simulink model "blance_leg2_RPY"  (R2023a)
settings: Solver=VariableStepAuto  StartTime=0.0  StopTime=10  MaxStep=0.0050000000000000001  RelTol=5.0000000000000002e-05  AbsTol=9.9999999999999995e-07
InitFcn:
  | addpath(fileparts(get_param(bdroot,'FileName')));
  | apply_config(bdroot);
model workspace (MAT data in the model file):
  L_length_ref : timeseries (value not decoded)
  L_v_ref : timeseries (value not decoded)
  R_length_ref : timeseries (value not decoded)
  R_v_ref : timeseries (value not decoded)
  runScenario_cfg_override = []
  wheel_speed_compensation = 1
values from neighbouring files (symbols this model uses):
  K = cachedK    [configured_lqr_gain.m]    (also in get_k_length.m = lqr(A,B,Q,R); matlab.mat = [-1.73670717704  -0.157075032659  -0.691811333866  -0.787613)
  N = NM + mp*diff(x + L*sin(theta),t,2)    [get_k_length.m]
  s = sin(phi3 - phi2)    [five_bar_geometry_rm.m]
undefined symbols (not defined in the file or in its folder): X, Y, Z
libraries: sm_lib x82, nesl_utility x35, slpidlib x2
(part 3 of 3)

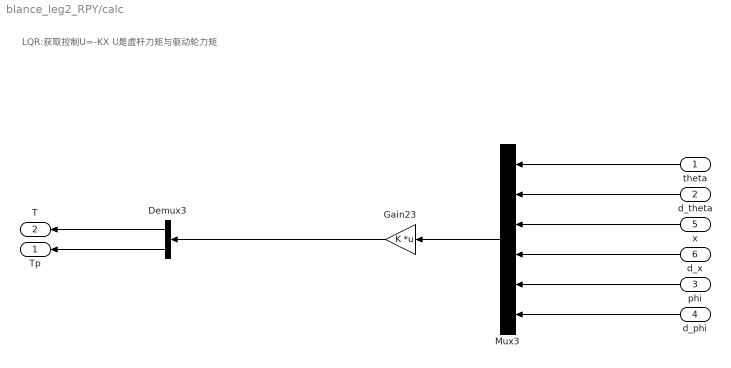
== system blance_leg2_RPY/calc ==
  note: LQR:获取控制U=-KX
      | U是虚杆力矩与驱动轮力矩
  theta : Inport
  d_theta : Inport  Port=2
  phi : Inport  Port=3
  d_phi : Inport  Port=4
  x : Inport  Port=5
  d_x : Inport  Port=6
  Demux3 : Demux  Outputs=2
  Gain23 : Gain  Gain=K  Multiplication=Matrix(K*u) (u vector)
  Mux3 : Mux  Inputs=6
  Tp : Outport
  T : Outport  Port=2
  wires:
  Demux3/1 -> T/1
  Demux3/2 -> Tp/1
  Mux3/1 -> Gain23/1
  theta/1 -> Mux3/1
  d_theta/1 -> Mux3/2
  x/1 -> Mux3/3
  d_x/1 -> Mux3/4
  phi/1 -> Mux3/5
  d_phi/1 -> Mux3/6
  Gain23/1 -> Demux3/1

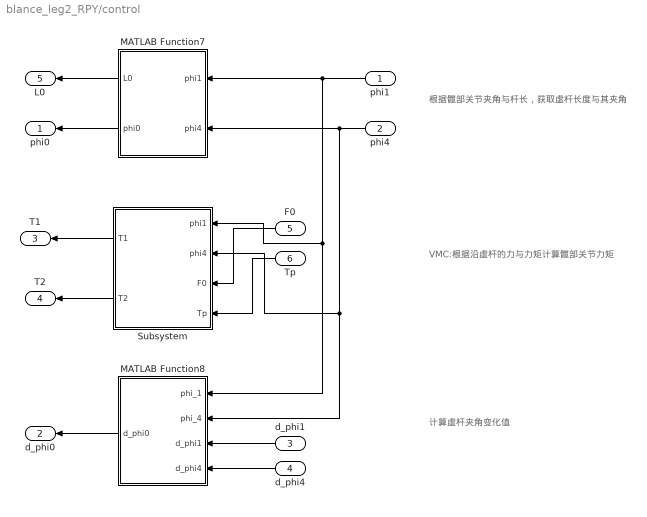
== system blance_leg2_RPY/control ==
  note: 计算虚杆夹角变化值
  note: VMC:根据沿虚杆的力与力矩计算髋部关节力矩
  note: 根据髋部关节夹角与杆长，获取虚杆长度与其夹角
  phi1 : Inport
  phi4 : Inport  Port=2
  d_phi1 : Inport  Port=3
  d_phi4 : Inport  Port=4
  F0 : Inport  Port=5
  Tp : Inport  Port=6
  MATLAB Function7 : MATLAB Function  TreatAsAtomicUnit=on
  MATLAB Function8 : MATLAB Function  TreatAsAtomicUnit=on
  Subsystem : Subsystem
  phi0 : Outport
  d_phi0 : Outport  Port=2
  T1 : Outport  Port=3
  T2 : Outport  Port=4
  L0 : Outport  Port=5
  wires:
  MATLAB Function7/2(phi0) -> phi0/1
  MATLAB Function8/1(d_phi0) -> d_phi0/1
  d_phi4/1 -> MATLAB Function8/4(d_phi4)
  d_phi1/1 -> MATLAB Function8/3(d_phi1)
  MATLAB Function7/1(L0) -> L0/1
  phi4/1 -> MATLAB Function7/2(phi4), Subsystem/2(phi4), MATLAB Function8/2(phi_4)
  phi1/1 -> MATLAB Function7/1(phi1), MATLAB Function8/1(phi_1), Subsystem/1(phi1)
  F0/1 -> Subsystem/3(F0)
  Tp/1 -> Subsystem/4(Tp)
  Subsystem/1(T1) -> T1/1
  Subsystem/2(T2) -> T2/1

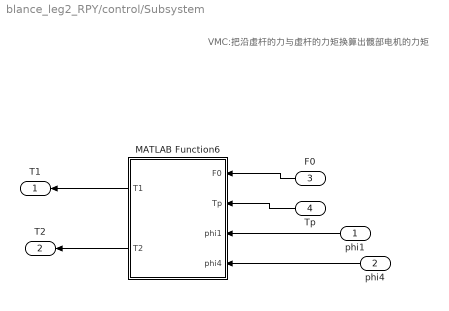
== system blance_leg2_RPY/control/Subsystem ==
  note: VMC:把沿虚杆的力与虚杆的力矩换算出髋部电机的力矩
  phi1 : Inport
  phi4 : Inport  Port=2
  F0 : Inport  Port=3
  Tp : Inport  Port=4
  MATLAB Function6 : MATLAB Function  TreatAsAtomicUnit=on
  T1 : Outport
  T2 : Outport  Port=2
  wires:
  phi1/1 -> MATLAB Function6/3(phi1)
  phi4/1 -> MATLAB Function6/4(phi4)
  Tp/1 -> MATLAB Function6/2(Tp)
  MATLAB Function6/1(T1) -> T1/1
  F0/1 -> MATLAB Function6/1(F0)
  MATLAB Function6/2(T2) -> T2/1

== matlab function blance_leg2_RPY/Subsystem4/MATLAB Function11 ==
  data: d_phi0 output; phi_1 input; phi_4 input; d_phi1 input; d_phi4 input
function d_phi0 = fcn(phi_1,phi_4,d_phi1,d_phi4)
   
    l5=0.10;%AE长度
    l1=0.12;
    l2=0.18;
    l3=0.18;
    l4=0.12;
    
    d_phi0 = (d_phi1*((l1*cos(phi_1) + (2*l2*cos(2*atan(((4*l2^2*(l1*sin(phi_1) - l4*sin(phi_4))^2 - ((l1*sin(phi_1) - l4*sin(phi_4))^2 + (l5 - l1*cos(phi_1) + l4*cos(phi_4))^2 + l2^2 - l3^2)^2 + 4*l2^2*(l5 - l1*cos(phi_1) + l4*cos(phi_4))^2)^(1/2) - 2*l2*(l1*sin(phi_1) - l4*sin(phi_4)))/((l1*sin(phi_1) - l4*sin(phi_4))^2 + (l5 - l1*cos(phi_1) + l4*cos(phi_4))^2 + l2^2 - l3^2 + 2*l2*(l5 - l1*cos(phi_1) + l4*cos(phi_4)))))*(((8*l1*l2^2*cos(phi_1)*(l1*sin(phi_1) - l4*sin(phi_4)) - 2*(2*l1*cos(phi_1)*(l1*sin(phi_1) - l4*sin(phi_4)) + 2*l1*sin(phi_1)*(l5 - l1*cos(phi_1) + l4*cos(phi_4)))*((l1*sin(phi_1) - l4*sin(phi_4))^2 + (l5 - l1*cos(phi_1) + l4*cos(phi_4))^2 + l2^2 - l3^2) + 8*l1*l2^2*sin(phi_1)*(l5 - l1*cos(phi_1) + l4*cos(phi_4)))/(2*(4*l2^2*(l1*sin(phi_1) - l4*sin(phi_4))^2 - ((l1*sin(phi_1) - l4*sin(phi_4))^2 + (l5 - l1*cos(phi_1) + l4*cos(phi_4))^2 + l2^2 - l3^2)^2 + 4*l2^2*(l5 - l1*cos(phi_1) + l4*cos(phi_4))^2)^(1/2)) - 2*l1*l2*cos(phi_1))/((l1*sin(phi_1) - l4*sin(phi_4))^2 + (l5 - l1*cos(phi_1) + l4*cos(phi_4))^2 + l2^2 - l3^2 + 2*l2*(l5 - l1*cos(phi_1) + l4*cos(phi_4))) - (((4*l2^2*(l1*sin(phi_1) - l4*sin(phi_4))^2 - ((l1*sin(phi_1) - l4*sin(phi_4))^2 + (l5 - l1*cos(phi_1) + l4*cos(phi_4))^2 + l2^2 - l3^2)^2 + 4*l2^2*(l5 - l1*cos(phi_1) + l4*cos(phi_4))^2)^(1/2) - 2*l2*(l1*sin(phi_1) - l4*sin(phi_4)))*(2*l1*l2*sin(phi_1) + 2*l1*cos(phi_1)*(l1*sin(phi_1) - l4*sin(phi_4)) + 2*l1*sin(phi_1)*(l5 - l1*cos(phi_1) + l4*cos(phi_4))))/((l1*sin(phi_1) - l4*sin(phi_4))^2 + (l5 - l1*cos(phi_1) + l4*cos(phi_4))^2 + l2^2 - l3^2 + 2*l2*(l5 - l1*cos(phi_1) + l4*cos(phi_4)))^2))/(((4*l2^2*(l1*sin(phi_1) - l4*sin(phi_4))^2 - ((l1*sin(phi_1) - l4*sin(phi_4))^2 + (l5 - l1*cos(phi_1) + l4*cos(phi_4))^2 + l2^2 - l3^2)^2 + 4*l2^2*(l5 - l1*cos(phi_1) + l4*cos(phi_4))^2)^(1/2) - 2*l2*(l1*sin(phi_1) - l4*sin(phi_4)))^2/((l1*sin(phi_1) - l4*sin(phi_4))^2 + (l5 - l1*cos(phi_1) + l4*cos(phi_4))^2 + l2^2 - l3^2 + 2*l2*(l5 - l1*cos(phi_1) + l4*cos(phi_4)))^2 + 1))/(l2*cos(2*atan(((4*l2^2*(l1*sin(phi_1) - l4*sin(phi_4))^2 - ((l1*sin(phi_1) - l4*sin(phi_4))^2 + (l5 - l1*cos(phi_1) + l4*cos(phi_4))^2 + l2^2 - l3^2)^2 + 4*l2^2*(l5 - l1*cos(phi_1) + l4*cos(phi_4))^2)^(1/2) - 2*l2*(l1*sin(phi_1) - l4*sin(phi_4)))/((l1*sin(phi_1) - l4*sin(phi_4))^2 + (l5 - l1*cos(phi_1) + l4*cos(phi_4))^2 + l2^2 - l3^2 + 2*l2*(l5 - l1*cos(phi_1) + l4*cos(phi_4))))) - l5/2 + l1*cos(phi_1)) + ((l2*sin(2*atan(((4*l2^2*(l1*sin(phi_1) - l4*sin(phi_4))^2 - ((l1*sin(phi_1) - l4*sin(phi_4))^2 + (l5 - l1*cos(phi_1) + l4*cos(phi_4))^2 + l2^2 - l3^2)^2 + 4*l2^2*(l5 - l1*cos(phi_1) + l4*cos(phi_4))^2)^(1/2) - 2*l2*(l1*sin(phi_1) - l4*sin(phi_4)))/((l1*sin(phi_1) - l4*sin(phi_4))^2 + (l5 - l1*cos(phi_1) + l4*cos(phi_4))^2 + l2^2 - l3^2 + 2*l2*(l5 - l1*cos(phi_1) + l4*cos(phi_4))))) + l1*sin(phi_1))*(l1*sin(phi_1) + (2*l2*sin(2*atan(((4*l2^2*(l1*sin(phi_1) - l4*sin(phi_4))^2 - ((l1*sin(phi_1) - l4*sin(phi_4))^2 + (l5 - l1*cos(phi_1) + l4*cos(phi_4))^2 + l2^2 - l3^2)^2 + 4*l2^2*(l5 - l1*cos(phi_1) + l4*cos(phi_4))^2)^(1/2) - 2*l2*(l1*sin(phi_1) - l4*sin(phi_4)))/((l1*sin(phi_1) - l4*sin(phi_4))^2 + (l5 - l1*cos(phi_1) + l4*cos(phi_4))^2 + l2^2 - l3^2 + 2*l2*(l5 - l1*cos(phi_1) + l4*cos(phi_4)))))*(((8*l1*l2^2*cos(phi_1)*(l1*sin(phi_1) - l4*sin(phi_4)) - 2*(2*l1*cos(phi_1)*(l1*sin(phi_1) - l4*sin(phi_4)) + 2*l1*sin(phi_1)*(l5 - l1*cos(phi_1) + l4*cos(phi_4)))*((l1*sin(phi_1) - l4*sin(phi_4))^2 + (l5 - l1*cos(phi_1) + l4*cos(phi_4))^2 + l2^2 - l3^2) + 8*l1*l2^2*sin(phi_1)*(l5 - l1*cos(phi_1) + l4*cos(phi_4)))/(2*(4*l2^2*(l1*sin(phi_1) - l4*sin(phi_4))^2 - ((l1*sin(phi_1) - l4*sin(phi_4))^2 + (l5 - l1*cos(phi_1) + l4*cos(phi_4))^2 + l2^2 - l3^2)^2 + 4*l2^2*(l5 - l1*cos(phi_1) + l4*cos(phi_4))^2)^(1/2)) - 2*l1*l2*cos(phi_1))/((l1*sin(phi_1) - l4*sin(phi_4))^2 + (l5 - l1*cos(phi_1) + l4*cos(phi_4))^2 + l2^2 - l3^2 + 2*l2*(l5 - l1*cos(phi_1) + l4*cos(phi_4))) - (((4*l2^2*(l1*sin(phi_1) - l4*sin(phi_4))^2 - ((l1*sin(phi_1) - l4*sin(phi_4))^2 + (l5 - l1*cos(phi_1) + l4*cos(phi_4))^2 + l2^2 - l3^2)^2 + 4*l2^2*(l5 - l1*cos(phi_1) + l4*cos(phi_4))^2)^(1/2) - 2*l2*(l1*sin(phi_1) - l4*sin(phi_4)))*(2*l1*l2*sin(phi_1) + 2*l1*cos(phi_1)*(l1*sin(phi_1) - l4*sin(phi_4)) + 2*l1*sin(phi_1)*(l5 - l1*cos(phi_1) + l4*cos(phi_4))))/((l1*sin(phi_1) - l4*sin(phi_4))^2 + (l5 - l1*cos(phi_1) + l4*cos(phi_4))^2 + l2^2 - l3^2 + 2*l2*(l5 - l1*cos(phi_1) + l4*cos(phi_4)))^2))/(((4*l2^2*(l1*sin(phi_1) - l4*sin(phi_4))^2 - ((l1*sin(phi_1) - l4*sin(phi_4))^2 + (l5 - l1*cos(phi_1) + l4*cos(phi_4))^2 + l2^2 - l3^2)^2 + 4*l2^2*(l5 - l1*cos(phi_1) + l4*cos(phi_4))^2)^(1/2) - 2*l2*(l1*sin(phi_1) - l4*sin(phi_4)))^2/((l1*sin(phi_1) - l4*sin(phi_4))^2 + (l5 - l1*cos(phi_1) + l4*cos(phi_4))^2 + l2^2 - l3^2 + 2*l2*(l5 - l1*cos(phi_1) + l4*cos(phi_4)))^2 + 1)))/(l2*cos(2*atan(((4*l2^2*(l1*sin(phi_1) - l4*sin(phi_4))^2 - ((l1*sin(phi_1) - l4*sin(phi_4))^2 + (l5 - l1*cos(phi_1) + l4*cos(phi_4))^2 + l2^2 - l3^2)^2 + 4*l2^2*(l5 - l1*cos(phi_1) + l4*cos(phi_4))^2)^(1/2) - 2*l2*(l1*sin(phi_1) - l4*sin(phi_4)))/((l1*sin(phi_1) - l4*sin(phi_4))^2 + (l5 - l1*cos(phi_1) + l4*cos(phi_4))^2 + l2^2 - l3^2 + 2*l2*(l5 - l1*cos(phi_1) + l4*cos(phi_4))))) - l5/2 + l1*cos(phi_1))^2))/((l2*sin(2*atan(((4*l2^2*(l1*sin(phi_1) - l4*sin(phi_4))^2 - ((l1*sin(phi_1) - l4*sin(phi_4))^2 + (l5 - l1*cos(phi_1) + l4*cos(phi_4))^2 + l2^2 - l3^2)^2 + 4*l2^2*(l5 - l1*cos(phi_1) + l4*cos(phi_4))^2)^(1/2) - 2*l2*(l1*sin(phi_1) - l4*sin(phi_4)))/((l1*sin(phi_1) - l4*sin(phi_4))^2 + (l5 - l1*cos(phi_1) + l4*cos(phi_4))^2 + l2^2 - l3^2 + 2*l2*(l5 - l1*cos(phi_1) + l4*cos(phi_4))))) + l1*sin(phi_1))^2/(l2*cos(2*atan(((4*l2^2*(l1*sin(phi_1) - l4*sin(phi_4))^2 - ((l1*sin(phi_1) - l4*sin(phi_4))^2 + (l5 - l1*cos(phi_1) + l4*cos(phi_4))^2 + l2^2 - l3^2)^2 + 4*l2^2*(l5 - l1*cos(phi_1) + l4*cos(phi_4))^2)^(1/2) - 2*l2*(l1*sin(phi_1) - l4*sin(phi_4)))/((l1*sin(phi_1) - l4*sin(phi_4))^2 + (l5 - l1*cos(phi_1) + l4*cos(phi_4))^2 + l2^2 - l3^2 + 2*l2*(l5 - l1*cos(phi_1) + l4*cos(phi_4))))) - l5/2 + l1*cos(phi_1))^2 + 1) - (d_phi4*((2*l2*cos(2*atan(((4*l2^2*(l1*sin(phi_1) - l4*sin(phi_4))^2 - ((l1*sin(phi_1) - l4*sin(phi_4))^2 + (l5 - l1*cos(phi_1) + l4*cos(phi_4))^2 + l2^2 - l3^2)^2 + 4*l2^2*(l5 - l1*cos(phi_1) + l4*cos(phi_4))^2)^(1/2) - 2*l2*(l1*sin(phi_1) - l4*sin(phi_4)))/((l1*sin(phi_1) - l4*sin(phi_4))^2 + (l5 - l1*cos(phi_1) + l4*cos(phi_4))^2 + l2^2 - l3^2 + 2*l2*(l5 - l1*cos(phi_1) + l4*cos(phi_4)))))*(((8*l2^2*l4*cos(phi_4)*(l1*sin(phi_1) - l4*sin(phi_4)) - 2*(2*l4*cos(phi_4)*(l1*sin(phi_1) - l4*sin(phi_4)) + 2*l4*sin(phi_4)*(l5 - l1*cos(phi_1) + l4*cos(phi_4)))*((l1*sin(phi_1) - l4*sin(phi_4))^2 + (l5 - l1*cos(phi_1) + l4*cos(phi_4))^2 + l2^2 - l3^2) + 8*l2^2*l4*sin(phi_4)*(l5 - l1*cos(phi_1) + l4*cos(phi_4)))/(2*(4*l2^2*(l1*sin(phi_1) - l4*sin(phi_4))^2 - ((l1*sin(phi_1) - l4*sin(phi_4))^2 + (l5 - l1*cos(phi_1) + l4*cos(phi_4))^2 + l2^2 - l3^2)^2 + 4*l2^2*(l5 - l1*cos(phi_1) + l4*cos(phi_4))^2)^(1/2)) - 2*l2*l4*cos(phi_4))/((l1*sin(phi_1) - l4*sin(phi_4))^2 + (l5 - l1*cos(phi_1) + l4*cos(phi_4))^2 + l2^2 - l3^2 + 2*l2*(l5 - l1*cos(phi_1) + l4*cos(phi_4))) - (((4*l2^2*(l1*sin(phi_1) - l4*sin(phi_4))^2 - ((l1*sin(phi_1) - l4*sin(phi_4))^2 + (l5 - l1*cos(phi_1) + l4*cos(phi_4))^2 + l2^2 - l3^2)^2 + 4*l2^2*(l5 - l1*cos(phi_1) + l4*cos(phi_4))^2)^(1/2) - 2*l2*(l1*sin(phi_1) - l4*sin(phi_4)))*(2*l2*l4*sin(phi_4) + 2*l4*cos(phi_4)*(l1*sin(phi_1) - l4*sin(phi_4)) + 2*l4*sin(phi_4)*(l5 - l1*cos(phi_1) + l4*cos(phi_4))))/((l1*sin(phi_1) - l4*sin(phi_4))^2 + (l5 - l1*cos(phi_1) + l4*cos(phi_4))^2 + l2^2 - l3^2 + 2*l2*(l5 - l1*cos(phi_1) + l4*cos(phi_4)))^2))/((((4*l2^2*(l1*sin(phi_1) - l4*sin(phi_4))^2 - ((l1*sin(phi_1) - l4*sin(phi_4))^2 + (l5 - l1*cos(phi_1) + l4*cos(phi_4))^2 + l2^2 - l3^2)^2 + 4*l2^2*(l5 - l1*cos(phi_1) + l4*cos(phi_4))^2)^(1/2) - 2*l2*(l1*sin(phi_1) - l4*sin(phi_4)))^2/((l1*sin(phi_1) - l4*sin(phi_4))^2 + (l5 - l1*cos(phi_1) + l4*cos(phi_4))^2 + l2^2 - l3^2 + 2*l2*(l5 - l1*cos(phi_1) + l4*cos(phi_4)))^2 + 1)*(l2*cos(2*atan(((4*l2^2*(l1*sin(phi_1) - l4*sin(phi_4))^2 - ((l1*sin(phi_1) - l4*sin(phi_4))^2 + (l5 - l1*cos(phi_1) + l4*cos(phi_4))^2 + l2^2 - l3^2)^2 + 4*l2^2*(l5 - l1*cos(phi_1) + l4*cos(phi_4))^2)^(1/2) - 2*l2*(l1*sin(phi_1) - l4*sin(phi_4)))/((l1*sin(phi_1) - l4*sin(phi_4))^2 + (l5 - l1*cos(phi_1) + l4*cos(phi_4))^2 + l2^2 - l3^2 + 2*l2*(l5 - l1*cos(phi_1) + l4*cos(phi_4))))) - l5/2 + l1*cos(phi_1))) + (2*l2*sin(2*atan(((4*l2^2*(l1*sin(phi_1) - l4*sin(phi_4))^2 - ((l1*sin(phi_1) - l4*sin(phi_4))^2 + (l5 - l1*cos(phi_1) + l4*cos(phi_4))^2 + l2^2 - l3^2)^2 + 4*l2^2*(l5 - l1*cos(phi_1) + l4*cos(phi_4))^2)^(1/2) - 2*l2*(l1*sin(phi_1) - l4*sin(phi_4)))/((l1*sin(phi_1) - l4*sin(phi_4))^2 + (l5 - l1*cos(phi_1) + l4*cos(phi_4))^2 + l2^2 - l3^2 + 2*l2*(l5 - l1*cos(phi_1) + l4*cos(phi_4)))))*(l2*sin(2*atan(((4*l2^2*(l1*sin(phi_1) - l4*sin(phi_4))^2 - ((l1*sin(phi_1) - l4*sin(phi_4))^2 + (l5 - l1*cos(phi_1) + l4*cos(phi_4))^2 + l2^2 - l3^2)^2 + 4*l2^2*(l5 - l1*cos(phi_1) + l4*cos(phi_4))^2)^(1/2) - 2*l2*(l1*sin(phi_1) - l4*sin(phi_4)))/((l1*sin(phi_1) - l4*sin(phi_4))^2 + (l5 - l1*cos(phi_1) + l4*cos(phi_4))^2 + l2^2 - l3^2 + 2*l2*(l5 - l1*cos(phi_1) + l4*cos(phi_4))))) + l1*sin(phi_1))*(((8*l2^2*l4*cos(phi_4)*(l1*sin(phi_1) - l4*sin(phi_4)) - 2*(2*l4*cos(phi_4)*(l1*sin(phi_1) - l4*sin(phi_4)) + 2*l4*sin(phi_4)*(l5 - l1*cos(phi_1) + l4*cos(phi_4)))*((l1*sin(phi_1) - l4*sin(phi_4))^2 + (l5 - l1*cos(phi_1) + l4*cos(phi_4))^2 + l2^2 - l3^2) + 8*l2^2*l4*sin(phi_4)*(l5 - l1*cos(phi_1) + l4*cos(phi_4)))/(2*(4*l2^2*(l1*sin(phi_1) - l4*sin(phi_4))^2 - ((l1*sin(phi_1) - l4*sin(phi_4))^2 + (l5 - l1*cos(phi_1) + l4*cos(phi_4))^2 + l2^2 - l3^2)^2 + 4*l2^2*(l5 - l1*cos(phi_1) + l4*cos(phi_4))^2)^(1/2)) - 2*l2*l4*cos(phi_4))/((l1*sin(phi_1) - l4*sin(phi_4))^2 + (l5 - l1*cos(phi_1) + l4*cos(phi_4))^2 + l2^2 - l3^2 + 2*l2*(l5 - l1*cos(phi_1) + l4*cos(phi_4))) - (((4*l2^2*(l1*sin(phi_1) - l4*sin(phi_4))^2 - ((l1*sin(phi_1) - l4*sin(phi_4))^2 + (l5 - l1*cos(phi_1) + l4*cos(phi_4))^2 + l2^2 - l3^2)^2 + 4*l2^2*(l5 - l1*cos(phi_1) + l4*cos(phi_4))^2)^(1/2) - 2*l2*(l1*sin(phi_1) - l4*sin(phi_4)))*(2*l2*l4*sin(phi_4) + 2*l4*cos(phi_4)*(l1*sin(phi_1) - l4*sin(phi_4)) + 2*l4*sin(phi_4)*(l5 - l1*cos(phi_1) + l4*cos(phi_4))))/((l1*sin(phi_1) - l4*sin(phi_4))^2 + (l5 - l1*cos(phi_1) + l4*cos(phi_4))^2 + l2^2 - l3^2 + 2*l2*(l5 - l1*cos(phi_1) + l4*cos(phi_4)))^2))/((((4*l2^2*(l1*sin(phi_1) - l4*sin(phi_4))^2 - ((l1*sin(phi_1) - l4*sin(phi_4))^2 + (l5 - l1*cos(phi_1) + l4*cos(phi_4))^2 + l2^2 - l3^2)^2 + 4*l2^2*(l5 - l1*cos(phi_1) + l4*cos(phi_4))^2)^(1/2) - 2*l2*(l1*sin(phi_1) - l4*sin(phi_4)))^2/((l1*sin(phi_1) - l4*sin(phi_4))^2 + (l5 - l1*cos(phi_1) + l4*cos(phi_4))^2 + l2^2 - l3^2 + 2*l2*(l5 - l1*cos(phi_1) + l4*cos(phi_4)))^2 + 1)*(l2*cos(2*atan(((4*l2^2*(l1*sin(phi_1) - l4*sin(phi_4))^2 - ((l1*sin(phi_1) - l4*sin(phi_4))^2 + (l5 - l1*cos(phi_1) + l4*cos(phi_4))^2 + l2^2 - l3^2)^2 + 4*l2^2*(l5 - l1*cos(phi_1) + l4*cos(phi_4))^2)^(1/2) - 2*l2*(l1*sin(phi_1) - l4*sin(phi_4)))/((l1*sin(phi_1) - l4*sin(phi_4))^2 + (l5 - l1*cos(phi_1) + l4*cos(phi_4))^2 + l2^2 - l3^2 + 2*l2*(l5 - l1*cos(phi_1) + l4*cos(phi_4))))) - l5/2 + l1*cos(phi_1))^2)))/((l2*sin(2*atan(((4*l2^2*(l1*sin(phi_1) - l4*sin(phi_4))^2 - ((l1*sin(phi_1) - l4*sin(phi_4))^2 + (l5 - l1*cos(phi_1) + l4*cos(phi_4))^2 + l2^2 - l3^2)^2 + 4*l2^2*(l5 - l1*cos(phi_1) + l4*cos(phi_4))^2)^(1/2) - 2*l2*(l1*sin(phi_1) - l4*sin(phi_4)))/((l1*sin(phi_1) - l4*sin(phi_4))^2 + (l5 - l1*cos(phi_1) + l4*cos(phi_4))^2 + l2^2 - l3^2 + 2*l2*(l5 - l1*cos(phi_1) + l4*cos(phi_4))))) + l1*sin(phi_1))^2/(l2*cos(2*atan(((4*l2^2*(l1*sin(phi_1) - l4*sin(phi_4))^2 - ((l1*sin(phi_1) - l4*sin(phi_4))^2 + (l5 - l1*cos(phi_1) + l4*cos(phi_4))^2 + l2^2 - l3^2)^2 + 4*l2^2*(l5 - l1*cos(phi_1) + l4*cos(phi_4))^2)^(1/2) - 2*l2*(l1*sin(phi_1) - l4*sin(phi_4)))/((l1*sin(phi_1) - l4*sin(phi_4))^2 + (l5 - l1*cos(phi_1) + l4*cos(phi_4))^2 + l2^2 - l3^2 + 2*l2*(l5 - l1*cos(phi_1) + l4*cos(phi_4))))) - l5/2 + l1*cos(phi_1))^2 + 1);
end
    % syms phi_0 phi_1 phi_2 phi_4 l1 l2 l3 l4 l5 L0 d_phi1 d_phi4
    % 
    % XD=l5+l4*cos(phi_4);
    % YD=l4*sin(phi_4);
    % XB=l1*cos(phi_1);
    % YB=l1*sin(phi_1);
    % A0=2*l2*(XD-XB);
    % B0=2*l2*(YD-YB);
    % lBD=sqrt((XD-XB)^2+(YD-YB)^2);
    % C0=l2^2+lBD^2-l3^2;
    % phi_2=2*atan((B0+sqrt(A0^2+B0^2-C0^2))/(A0+C0));
    % XC=XB+l2*cos(phi_2);
    % YC=YB+l2*sin(phi_2);
    % L0=sqrt((XC-l5/2)^2+YC^2);
    % phi_0=atan(YC/(XC-l5/2));
    % 
    % J=jacobian([L0;phi_0],[phi_1;phi_4]);
    % phi0_dot = J(2,1)*d_phi1 +J(2,2)*d_phi4

    % jacobian函数无法在simulink中使用，故直接使用jacobian函数的最终结果

== matlab function blance_leg2_RPY/control/Subsystem/MATLAB Function6 ==
  data: F0 input; T1 output; Tp input; phi1 input; phi4 input; T2 output
function [T1,T2] = VMC_calc(F0,Tp,phi1,phi4)

    l5=0.10;%AE长度
    l1=0.12;
    l2=0.18;
    l3=0.18;
    l4=0.12;

YD = l4*sin(phi4);
YB = l1*sin(phi1);
XD = l5 + l4*cos(phi4);
XB = l1*cos(phi1); 
lBD = sqrt((XD - XB)*(XD - XB) + (YD - YB)*(YD - YB));
A0 = 2*l2*(XD - XB);
B0 = 2*l2*(YD - YB);
C0 = l2*l2 + lBD*lBD - l3*l3;
phi2 = 2*atan2((B0 + sqrt(A0*A0 + B0*B0 - C0*C0)),A0 + C0);
phi3 = atan2(YB-YD+l2*sin(phi2),XB-XD+l2*cos(phi2));
XC = l1*cos(phi1) + l2*cos(phi2);
YC = l1*sin(phi1) + l2*sin(phi2);
L0 = sqrt((XC - l5/2)*(XC - l5/2) + YC*YC);
phi0 = atan2(YC,XC - l5/2);
j11 = (l1*sin(phi0-phi3)*sin(phi1-phi2))/sin(phi3-phi2);
j12 = (l1*cos(phi0-phi3)*sin(phi1-phi2))/(L0*sin(phi3-phi2));
j21 = (l4*sin(phi0-phi2)*sin(phi3-phi4))/sin(phi3-phi2);
j22 = (l4*cos(phi0-phi2)*sin(phi3-phi4))/(L0*sin(phi3-phi2));
J = [j11 j12; j21 j22];
F = [F0;Tp];
T = J * F;
T1 = T(1,1);
T2 = T(2,1);

end

== matlab function blance_leg2_RPY/control/MATLAB Function7 ==
  data: L0 output; phi1 input; phi4 input; phi0 output
function [L0,phi0] = fcn(phi1,phi4)
  
    l5=0.10;%AE长度
    l1=0.12;
    l2=0.18;
    l3=0.18;
    l4=0.12;
    
    YD = l4*sin(phi4);
    YB = l1*sin(phi1);
    XD = l5 + l4*cos(phi4);
    XB = l1*cos(phi1); 
    lBD = sqrt((XD - XB)*(XD - XB) + (YD - YB)*(YD - YB));
    A0 = 2*l2*(XD - XB);
    B0 = 2*l2*(YD - YB);
    C0 = l2*l2 + lBD*lBD - l3*l3;
    phi2 = 2*atan2((B0 + sqrt(A0*A0 + B0*B0 - C0*C0)),(A0 + C0));
    XC = l1*cos(phi1) + l2*cos(phi2);
    YC = l1*sin(phi1) + l2*sin(phi2);
    L0 = sqrt((XC - l5/2)*(XC - l5/2) + YC*YC);
    phi0=atan2(YC,(XC-l5/2));
end

== matlab function blance_leg2_RPY/control/MATLAB Function8 ==
  data: d_phi0 output; phi_1 input; phi_4 input; d_phi1 input; d_phi4 input
% 计算虚杆夹角变化值
function d_phi0 = fcn(phi_1,phi_4,d_phi1,d_phi4)
   
    l5=0.10;%AE长度
    l1=0.12;
    l2=0.18;
    l3=0.18;
    l4=0.12;
    
    d_phi0 = (d_phi1*((l1*cos(phi_1) + (2*l2*cos(2*atan(((4*l2^2*(l1*sin(phi_1) - l4*sin(phi_4))^2 - ((l1*sin(phi_1) - l4*sin(phi_4))^2 + (l5 - l1*cos(phi_1) + l4*cos(phi_4))^2 + l2^2 - l3^2)^2 + 4*l2^2*(l5 - l1*cos(phi_1) + l4*cos(phi_4))^2)^(1/2) - 2*l2*(l1*sin(phi_1) - l4*sin(phi_4)))/((l1*sin(phi_1) - l4*sin(phi_4))^2 + (l5 - l1*cos(phi_1) + l4*cos(phi_4))^2 + l2^2 - l3^2 + 2*l2*(l5 - l1*cos(phi_1) + l4*cos(phi_4)))))*(((8*l1*l2^2*cos(phi_1)*(l1*sin(phi_1) - l4*sin(phi_4)) - 2*(2*l1*cos(phi_1)*(l1*sin(phi_1) - l4*sin(phi_4)) + 2*l1*sin(phi_1)*(l5 - l1*cos(phi_1) + l4*cos(phi_4)))*((l1*sin(phi_1) - l4*sin(phi_4))^2 + (l5 - l1*cos(phi_1) + l4*cos(phi_4))^2 + l2^2 - l3^2) + 8*l1*l2^2*sin(phi_1)*(l5 - l1*cos(phi_1) + l4*cos(phi_4)))/(2*(4*l2^2*(l1*sin(phi_1) - l4*sin(phi_4))^2 - ((l1*sin(phi_1) - l4*sin(phi_4))^2 + (l5 - l1*cos(phi_1) + l4*cos(phi_4))^2 + l2^2 - l3^2)^2 + 4*l2^2*(l5 - l1*cos(phi_1) + l4*cos(phi_4))^2)^(1/2)) - 2*l1*l2*cos(phi_1))/((l1*sin(phi_1) - l4*sin(phi_4))^2 + (l5 - l1*cos(phi_1) + l4*cos(phi_4))^2 + l2^2 - l3^2 + 2*l2*(l5 - l1*cos(phi_1) + l4*cos(phi_4))) - (((4*l2^2*(l1*sin(phi_1) - l4*sin(phi_4))^2 - ((l1*sin(phi_1) - l4*sin(phi_4))^2 + (l5 - l1*cos(phi_1) + l4*cos(phi_4))^2 + l2^2 - l3^2)^2 + 4*l2^2*(l5 - l1*cos(phi_1) + l4*cos(phi_4))^2)^(1/2) - 2*l2*(l1*sin(phi_1) - l4*sin(phi_4)))*(2*l1*l2*sin(phi_1) + 2*l1*cos(phi_1)*(l1*sin(phi_1) - l4*sin(phi_4)) + 2*l1*sin(phi_1)*(l5 - l1*cos(phi_1) + l4*cos(phi_4))))/((l1*sin(phi_1) - l4*sin(phi_4))^2 + (l5 - l1*cos(phi_1) + l4*cos(phi_4))^2 + l2^2 - l3^2 + 2*l2*(l5 - l1*cos(phi_1) + l4*cos(phi_4)))^2))/(((4*l2^2*(l1*sin(phi_1) - l4*sin(phi_4))^2 - ((l1*sin(phi_1) - l4*sin(phi_4))^2 + (l5 - l1*cos(phi_1) + l4*cos(phi_4))^2 + l2^2 - l3^2)^2 + 4*l2^2*(l5 - l1*cos(phi_1) + l4*cos(phi_4))^2)^(1/2) - 2*l2*(l1*sin(phi_1) - l4*sin(phi_4)))^2/((l1*sin(phi_1) - l4*sin(phi_4))^2 + (l5 - l1*cos(phi_1) + l4*cos(phi_4))^2 + l2^2 - l3^2 + 2*l2*(l5 - l1*cos(phi_1) + l4*cos(phi_4)))^2 + 1))/(l2*cos(2*atan(((4*l2^2*(l1*sin(phi_1) - l4*sin(phi_4))^2 - ((l1*sin(phi_1) - l4*sin(phi_4))^2 + (l5 - l1*cos(phi_1) + l4*cos(phi_4))^2 + l2^2 - l3^2)^2 + 4*l2^2*(l5 - l1*cos(phi_1) + l4*cos(phi_4))^2)^(1/2) - 2*l2*(l1*sin(phi_1) - l4*sin(phi_4)))/((l1*sin(phi_1) - l4*sin(phi_4))^2 + (l5 - l1*cos(phi_1) + l4*cos(phi_4))^2 + l2^2 - l3^2 + 2*l2*(l5 - l1*cos(phi_1) + l4*cos(phi_4))))) - l5/2 + l1*cos(phi_1)) + ((l2*sin(2*atan(((4*l2^2*(l1*sin(phi_1) - l4*sin(phi_4))^2 - ((l1*sin(phi_1) - l4*sin(phi_4))^2 + (l5 - l1*cos(phi_1) + l4*cos(phi_4))^2 + l2^2 - l3^2)^2 + 4*l2^2*(l5 - l1*cos(phi_1) + l4*cos(phi_4))^2)^(1/2) - 2*l2*(l1*sin(phi_1) - l4*sin(phi_4)))/((l1*sin(phi_1) - l4*sin(phi_4))^2 + (l5 - l1*cos(phi_1) + l4*cos(phi_4))^2 + l2^2 - l3^2 + 2*l2*(l5 - l1*cos(phi_1) + l4*cos(phi_4))))) + l1*sin(phi_1))*(l1*sin(phi_1) + (2*l2*sin(2*atan(((4*l2^2*(l1*sin(phi_1) - l4*sin(phi_4))^2 - ((l1*sin(phi_1) - l4*sin(phi_4))^2 + (l5 - l1*cos(phi_1) + l4*cos(phi_4))^2 + l2^2 - l3^2)^2 + 4*l2^2*(l5 - l1*cos(phi_1) + l4*cos(phi_4))^2)^(1/2) - 2*l2*(l1*sin(phi_1) - l4*sin(phi_4)))/((l1*sin(phi_1) - l4*sin(phi_4))^2 + (l5 - l1*cos(phi_1) + l4*cos(phi_4))^2 + l2^2 - l3^2 + 2*l2*(l5 - l1*cos(phi_1) + l4*cos(phi_4)))))*(((8*l1*l2^2*cos(phi_1)*(l1*sin(phi_1) - l4*sin(phi_4)) - 2*(2*l1*cos(phi_1)*(l1*sin(phi_1) - l4*sin(phi_4)) + 2*l1*sin(phi_1)*(l5 - l1*cos(phi_1) + l4*cos(phi_4)))*((l1*sin(phi_1) - l4*sin(phi_4))^2 + (l5 - l1*cos(phi_1) + l4*cos(phi_4))^2 + l2^2 - l3^2) + 8*l1*l2^2*sin(phi_1)*(l5 - l1*cos(phi_1) + l4*cos(phi_4)))/(2*(4*l2^2*(l1*sin(phi_1) - l4*sin(phi_4))^2 - ((l1*sin(phi_1) - l4*sin(phi_4))^2 + (l5 - l1*cos(phi_1) + l4*cos(phi_4))^2 + l2^2 - l3^2)^2 + 4*l2^2*(l5 - l1*cos(phi_1) + l4*cos(phi_4))^2)^(1/2)) - 2*l1*l2*cos(phi_1))/((l1*sin(phi_1) - l4*sin(phi_4))^2 + (l5 - l1*cos(phi_1) + l4*cos(phi_4))^2 + l2^2 - l3^2 + 2*l2*(l5 - l1*cos(phi_1) + l4*cos(phi_4))) - (((4*l2^2*(l1*sin(phi_1) - l4*sin(phi_4))^2 - ((l1*sin(phi_1) - l4*sin(phi_4))^2 + (l5 - l1*cos(phi_1) + l4*cos(phi_4))^2 + l2^2 - l3^2)^2 + 4*l2^2*(l5 - l1*cos(phi_1) + l4*cos(phi_4))^2)^(1/2) - 2*l2*(l1*sin(phi_1) - l4*sin(phi_4)))*(2*l1*l2*sin(phi_1) + 2*l1*cos(phi_1)*(l1*sin(phi_1) - l4*sin(phi_4)) + 2*l1*sin(phi_1)*(l5 - l1*cos(phi_1) + l4*cos(phi_4))))/((l1*sin(phi_1) - l4*sin(phi_4))^2 + (l5 - l1*cos(phi_1) + l4*cos(phi_4))^2 + l2^2 - l3^2 + 2*l2*(l5 - l1*cos(phi_1) + l4*cos(phi_4)))^2))/(((4*l2^2*(l1*sin(phi_1) - l4*sin(phi_4))^2 - ((l1*sin(phi_1) - l4*sin(phi_4))^2 + (l5 - l1*cos(phi_1) + l4*cos(phi_4))^2 + l2^2 - l3^2)^2 + 4*l2^2*(l5 - l1*cos(phi_1) + l4*cos(phi_4))^2)^(1/2) - 2*l2*(l1*sin(phi_1) - l4*sin(phi_4)))^2/((l1*sin(phi_1) - l4*sin(phi_4))^2 + (l5 - l1*cos(phi_1) + l4*cos(phi_4))^2 + l2^2 - l3^2 + 2*l2*(l5 - l1*cos(phi_1) + l4*cos(phi_4)))^2 + 1)))/(l2*cos(2*atan(((4*l2^2*(l1*sin(phi_1) - l4*sin(phi_4))^2 - ((l1*sin(phi_1) - l4*sin(phi_4))^2 + (l5 - l1*cos(phi_1) + l4*cos(phi_4))^2 + l2^2 - l3^2)^2 + 4*l2^2*(l5 - l1*cos(phi_1) + l4*cos(phi_4))^2)^(1/2) - 2*l2*(l1*sin(phi_1) - l4*sin(phi_4)))/((l1*sin(phi_1) - l4*sin(phi_4))^2 + (l5 - l1*cos(phi_1) + l4*cos(phi_4))^2 + l2^2 - l3^2 + 2*l2*(l5 - l1*cos(phi_1) + l4*cos(phi_4))))) - l5/2 + l1*cos(phi_1))^2))/((l2*sin(2*atan(((4*l2^2*(l1*sin(phi_1) - l4*sin(phi_4))^2 - ((l1*sin(phi_1) - l4*sin(phi_4))^2 + (l5 - l1*cos(phi_1) + l4*cos(phi_4))^2 + l2^2 - l3^2)^2 + 4*l2^2*(l5 - l1*cos(phi_1) + l4*cos(phi_4))^2)^(1/2) - 2*l2*(l1*sin(phi_1) - l4*sin(phi_4)))/((l1*sin(phi_1) - l4*sin(phi_4))^2 + (l5 - l1*cos(phi_1) + l4*cos(phi_4))^2 + l2^2 - l3^2 + 2*l2*(l5 - l1*cos(phi_1) + l4*cos(phi_4))))) + l1*sin(phi_1))^2/(l2*cos(2*atan(((4*l2^2*(l1*sin(phi_1) - l4*sin(phi_4))^2 - ((l1*sin(phi_1) - l4*sin(phi_4))^2 + (l5 - l1*cos(phi_1) + l4*cos(phi_4))^2 + l2^2 - l3^2)^2 + 4*l2^2*(l5 - l1*cos(phi_1) + l4*cos(phi_4))^2)^(1/2) - 2*l2*(l1*sin(phi_1) - l4*sin(phi_4)))/((l1*sin(phi_1) - l4*sin(phi_4))^2 + (l5 - l1*cos(phi_1) + l4*cos(phi_4))^2 + l2^2 - l3^2 + 2*l2*(l5 - l1*cos(phi_1) + l4*cos(phi_4))))) - l5/2 + l1*cos(phi_1))^2 + 1) - (d_phi4*((2*l2*cos(2*atan(((4*l2^2*(l1*sin(phi_1) - l4*sin(phi_4))^2 - ((l1*sin(phi_1) - l4*sin(phi_4))^2 + (l5 - l1*cos(phi_1) + l4*cos(phi_4))^2 + l2^2 - l3^2)^2 + 4*l2^2*(l5 - l1*cos(phi_1) + l4*cos(phi_4))^2)^(1/2) - 2*l2*(l1*sin(phi_1) - l4*sin(phi_4)))/((l1*sin(phi_1) - l4*sin(phi_4))^2 + (l5 - l1*cos(phi_1) + l4*cos(phi_4))^2 + l2^2 - l3^2 + 2*l2*(l5 - l1*cos(phi_1) + l4*cos(phi_4)))))*(((8*l2^2*l4*cos(phi_4)*(l1*sin(phi_1) - l4*sin(phi_4)) - 2*(2*l4*cos(phi_4)*(l1*sin(phi_1) - l4*sin(phi_4)) + 2*l4*sin(phi_4)*(l5 - l1*cos(phi_1) + l4*cos(phi_4)))*((l1*sin(phi_1) - l4*sin(phi_4))^2 + (l5 - l1*cos(phi_1) + l4*cos(phi_4))^2 + l2^2 - l3^2) + 8*l2^2*l4*sin(phi_4)*(l5 - l1*cos(phi_1) + l4*cos(phi_4)))/(2*(4*l2^2*(l1*sin(phi_1) - l4*sin(phi_4))^2 - ((l1*sin(phi_1) - l4*sin(phi_4))^2 + (l5 - l1*cos(phi_1) + l4*cos(phi_4))^2 + l2^2 - l3^2)^2 + 4*l2^2*(l5 - l1*cos(phi_1) + l4*cos(phi_4))^2)^(1/2)) - 2*l2*l4*cos(phi_4))/((l1*sin(phi_1) - l4*sin(phi_4))^2 + (l5 - l1*cos(phi_1) + l4*cos(phi_4))^2 + l2^2 - l3^2 + 2*l2*(l5 - l1*cos(phi_1) + l4*cos(phi_4))) - (((4*l2^2*(l1*sin(phi_1) - l4*sin(phi_4))^2 - ((l1*sin(phi_1) - l4*sin(phi_4))^2 + (l5 - l1*cos(phi_1) + l4*cos(phi_4))^2 + l2^2 - l3^2)^2 + 4*l2^2*(l5 - l1*cos(phi_1) + l4*cos(phi_4))^2)^(1/2) - 2*l2*(l1*sin(phi_1) - l4*sin(phi_4)))*(2*l2*l4*sin(phi_4) + 2*l4*cos(phi_4)*(l1*sin(phi_1) - l4*sin(phi_4)) + 2*l4*sin(phi_4)*(l5 - l1*cos(phi_1) + l4*cos(phi_4))))/((l1*sin(phi_1) - l4*sin(phi_4))^2 + (l5 - l1*cos(phi_1) + l4*cos(phi_4))^2 + l2^2 - l3^2 + 2*l2*(l5 - l1*cos(phi_1) + l4*cos(phi_4)))^2))/((((4*l2^2*(l1*sin(phi_1) - l4*sin(phi_4))^2 - ((l1*sin(phi_1) - l4*sin(phi_4))^2 + (l5 - l1*cos(phi_1) + l4*cos(phi_4))^2 + l2^2 - l3^2)^2 + 4*l2^2*(l5 - l1*cos(phi_1) + l4*cos(phi_4))^2)^(1/2) - 2*l2*(l1*sin(phi_1) - l4*sin(phi_4)))^2/((l1*sin(phi_1) - l4*sin(phi_4))^2 + (l5 - l1*cos(phi_1) + l4*cos(phi_4))^2 + l2^2 - l3^2 + 2*l2*(l5 - l1*cos(phi_1) + l4*cos(phi_4)))^2 + 1)*(l2*cos(2*atan(((4*l2^2*(l1*sin(phi_1) - l4*sin(phi_4))^2 - ((l1*sin(phi_1) - l4*sin(phi_4))^2 + (l5 - l1*cos(phi_1) + l4*cos(phi_4))^2 + l2^2 - l3^2)^2 + 4*l2^2*(l5 - l1*cos(phi_1) + l4*cos(phi_4))^2)^(1/2) - 2*l2*(l1*sin(phi_1) - l4*sin(phi_4)))/((l1*sin(phi_1) - l4*sin(phi_4))^2 + (l5 - l1*cos(phi_1) + l4*cos(phi_4))^2 + l2^2 - l3^2 + 2*l2*(l5 - l1*cos(phi_1) + l4*cos(phi_4))))) - l5/2 + l1*cos(phi_1))) + (2*l2*sin(2*atan(((4*l2^2*(l1*sin(phi_1) - l4*sin(phi_4))^2 - ((l1*sin(phi_1) - l4*sin(phi_4))^2 + (l5 - l1*cos(phi_1) + l4*cos(phi_4))^2 + l2^2 - l3^2)^2 + 4*l2^2*(l5 - l1*cos(phi_1) + l4*cos(phi_4))^2)^(1/2) - 2*l2*(l1*sin(phi_1) - l4*sin(phi_4)))/((l1*sin(phi_1) - l4*sin(phi_4))^2 + (l5 - l1*cos(phi_1) + l4*cos(phi_4))^2 + l2^2 - l3^2 + 2*l2*(l5 - l1*cos(phi_1) + l4*cos(phi_4)))))*(l2*sin(2*atan(((4*l2^2*(l1*sin(phi_1) - l4*sin(phi_4))^2 - ((l1*sin(phi_1) - l4*sin(phi_4))^2 + (l5 - l1*cos(phi_1) + l4*cos(phi_4))^2 + l2^2 - l3^2)^2 + 4*l2^2*(l5 - l1*cos(phi_1) + l4*cos(phi_4))^2)^(1/2) - 2*l2*(l1*sin(phi_1) - l4*sin(phi_4)))/((l1*sin(phi_1) - l4*sin(phi_4))^2 + (l5 - l1*cos(phi_1) + l4*cos(phi_4))^2 + l2^2 - l3^2 + 2*l2*(l5 - l1*cos(phi_1) + l4*cos(phi_4))))) + l1*sin(phi_1))*(((8*l2^2*l4*cos(phi_4)*(l1*sin(phi_1) - l4*sin(phi_4)) - 2*(2*l4*cos(phi_4)*(l1*sin(phi_1) - l4*sin(phi_4)) + 2*l4*sin(phi_4)*(l5 - l1*cos(phi_1) + l4*cos(phi_4)))*((l1*sin(phi_1) - l4*sin(phi_4))^2 + (l5 - l1*cos(phi_1) + l4*cos(phi_4))^2 + l2^2 - l3^2) + 8*l2^2*l4*sin(phi_4)*(l5 - l1*cos(phi_1) + l4*cos(phi_4)))/(2*(4*l2^2*(l1*sin(phi_1) - l4*sin(phi_4))^2 - ((l1*sin(phi_1) - l4*sin(phi_4))^2 + (l5 - l1*cos(phi_1) + l4*cos(phi_4))^2 + l2^2 - l3^2)^2 + 4*l2^2*(l5 - l1*cos(phi_1) + l4*cos(phi_4))^2)^(1/2)) - 2*l2*l4*cos(phi_4))/((l1*sin(phi_1) - l4*sin(phi_4))^2 + (l5 - l1*cos(phi_1) + l4*cos(phi_4))^2 + l2^2 - l3^2 + 2*l2*(l5 - l1*cos(phi_1) + l4*cos(phi_4))) - (((4*l2^2*(l1*sin(phi_1) - l4*sin(phi_4))^2 - ((l1*sin(phi_1) - l4*sin(phi_4))^2 + (l5 - l1*cos(phi_1) + l4*cos(phi_4))^2 + l2^2 - l3^2)^2 + 4*l2^2*(l5 - l1*cos(phi_1) + l4*cos(phi_4))^2)^(1/2) - 2*l2*(l1*sin(phi_1) - l4*sin(phi_4)))*(2*l2*l4*sin(phi_4) + 2*l4*cos(phi_4)*(l1*sin(phi_1) - l4*sin(phi_4)) + 2*l4*sin(phi_4)*(l5 - l1*cos(phi_1) + l4*cos(phi_4))))/((l1*sin(phi_1) - l4*sin(phi_4))^2 + (l5 - l1*cos(phi_1) + l4*cos(phi_4))^2 + l2^2 - l3^2 + 2*l2*(l5 - l1*cos(phi_1) + l4*cos(phi_4)))^2))/((((4*l2^2*(l1*sin(phi_1) - l4*sin(phi_4))^2 - ((l1*sin(phi_1) - l4*sin(phi_4))^2 + (l5 - l1*cos(phi_1) + l4*cos(phi_4))^2 + l2^2 - l3^2)^2 + 4*l2^2*(l5 - l1*cos(phi_1) + l4*cos(phi_4))^2)^(1/2) - 2*l2*(l1*sin(phi_1) - l4*sin(phi_4)))^2/((l1*sin(phi_1) - l4*sin(phi_4))^2 + (l5 - l1*cos(phi_1) + l4*cos(phi_4))^2 + l2^2 - l3^2 + 2*l2*(l5 - l1*cos(phi_1) + l4*cos(phi_4)))^2 + 1)*(l2*cos(2*atan(((4*l2^2*(l1*sin(phi_1) - l4*sin(phi_4))^2 - ((l1*sin(phi_1) - l4*sin(phi_4))^2 + (l5 - l1*cos(phi_1) + l4*cos(phi_4))^2 + l2^2 - l3^2)^2 + 4*l2^2*(l5 - l1*cos(phi_1) + l4*cos(phi_4))^2)^(1/2) - 2*l2*(l1*sin(phi_1) - l4*sin(phi_4)))/((l1*sin(phi_1) - l4*sin(phi_4))^2 + (l5 - l1*cos(phi_1) + l4*cos(phi_4))^2 + l2^2 - l3^2 + 2*l2*(l5 - l1*cos(phi_1) + l4*cos(phi_4))))) - l5/2 + l1*cos(phi_1))^2)))/((l2*sin(2*atan(((4*l2^2*(l1*sin(phi_1) - l4*sin(phi_4))^2 - ((l1*sin(phi_1) - l4*sin(phi_4))^2 + (l5 - l1*cos(phi_1) + l4*cos(phi_4))^2 + l2^2 - l3^2)^2 + 4*l2^2*(l5 - l1*cos(phi_1) + l4*cos(phi_4))^2)^(1/2) - 2*l2*(l1*sin(phi_1) - l4*sin(phi_4)))/((l1*sin(phi_1) - l4*sin(phi_4))^2 + (l5 - l1*cos(phi_1) + l4*cos(phi_4))^2 + l2^2 - l3^2 + 2*l2*(l5 - l1*cos(phi_1) + l4*cos(phi_4))))) + l1*sin(phi_1))^2/(l2*cos(2*atan(((4*l2^2*(l1*sin(phi_1) - l4*sin(phi_4))^2 - ((l1*sin(phi_1) - l4*sin(phi_4))^2 + (l5 - l1*cos(phi_1) + l4*cos(phi_4))^2 + l2^2 - l3^2)^2 + 4*l2^2*(l5 - l1*cos(phi_1) + l4*cos(phi_4))^2)^(1/2) - 2*l2*(l1*sin(phi_1) - l4*sin(phi_4)))/((l1*sin(phi_1) - l4*sin(phi_4))^2 + (l5 - l1*cos(phi_1) + l4*cos(phi_4))^2 + l2^2 - l3^2 + 2*l2*(l5 - l1*cos(phi_1) + l4*cos(phi_4))))) - l5/2 + l1*cos(phi_1))^2 + 1);
end

    % syms phi_0 phi_1 phi_2 phi_4 l1 l2 l3 l4 l5 L0 d_phi1 d_phi4
    % 
    % XD=l5+l4*cos(phi_4);
    % YD=l4*sin(phi_4);
    % XB=l1*cos(phi_1);
    % YB=l1*sin(phi_1);
    % A0=2*l2*(XD-XB);
    % B0=2*l2*(YD-YB);
    % lBD=sqrt((XD-XB)^2+(YD-YB)^2);
    % C0=l2^2+lBD^2-l3^2;
    % phi_2=2*atan((B0+sqrt(A0^2+B0^2-C0^2))/(A0+C0));
    % XC=XB+l2*cos(phi_2);
    % YC=YB+l2*sin(phi_2);
    % L0=sqrt((XC-l5/2)^2+YC^2);
    % phi_0=atan(YC/(XC-l5/2));
    % 
    % J=jacobian([L0;phi_0],[phi_1;phi_4]);
    % phi0_dot = J(2,1)*d_phi1 +J(2,2)*d_phi4

    % jacobian函数无法在simulink中使用，故直接使用jacobian函数的最终结果

== matlab function blance_leg2_RPY/Subsystem4/MATLAB Function9 ==
  data: F0 input; T1 output; Tp input; phi1 input; phi4 input; T2 output
function [T1,T2] = VMC_calc(F0,Tp,phi1,phi4)

    l5=0.10;%AE长度
    l1=0.12;
    l2=0.18;
    l3=0.18;
    l4=0.12;

YD = l4*sin(phi4);
YB = l1*sin(phi1);
XD = l5 + l4*cos(phi4);
XB = l1*cos(phi1); 
lBD = sqrt((XD - XB)*(XD - XB) + (YD - YB)*(YD - YB));
A0 = 2*l2*(XD - XB);
B0 = 2*l2*(YD - YB);
C0 = l2*l2 + lBD*lBD - l3*l3;
phi2 = 2*atan2((B0 + sqrt(A0*A0 + B0*B0 - C0*C0)),A0 + C0);
phi3 = atan2(YB-YD+l2*sin(phi2),XB-XD+l2*cos(phi2));
XC = l1*cos(phi1) + l2*cos(phi2);
YC = l1*sin(phi1) + l2*sin(phi2);
L0 = sqrt((XC - l5/2)*(XC - l5/2) + YC*YC);
phi0 = atan2(YC,XC - l5/2);
j11 = (l1*sin(phi0-phi3)*sin(phi1-phi2))/sin(phi3-phi2);
j12 = (l1*cos(phi0-phi3)*sin(phi1-phi2))/(L0*sin(phi3-phi2));
j21 = (l4*sin(phi0-phi2)*sin(phi3-phi4))/sin(phi3-phi2);
j22 = (l4*cos(phi0-phi2)*sin(phi3-phi4))/(L0*sin(phi3-phi2));
J = [j11 j12; j21 j22];
F = [F0;Tp];
T = J * F;
T1 = T(1,1);
T2 = T(2,1);
end

== matlab function blance_leg2_RPY/Scenario References/Landing length reference ==
  settings: updateMethod=DISCRETE  sampleTime=0.001
  data: L_length_request input; L_length_ref output; R_length_request input; L_length_meas input; R_length_meas input; on_ground input; R_length_ref output
function [L_length_ref, R_length_ref] = fcn( ...
    L_length_request, R_length_request, L_length_meas, R_length_meas, on_ground)
% 以 1 ms 执行。启动时记录实测腿长；双轮稳定接地后才改变目标。
% 离地时保持最后一次有效目标，重新确认接地后再继续。
persistent initialized ground_samples L_ref R_ref
if isempty(initialized)
    initialized = false;
    ground_samples = 0;
    L_ref = 0.0831;
    R_ref = 0.0831;
end

if ~initialized
    if isfinite(L_length_meas) && isfinite(R_length_meas) ...
            && L_length_meas > 0 && R_length_meas > 0
        L_ref = L_length_meas;
        R_ref = R_length_meas;
        initialized = true;
    end
elseif on_ground
    % 连续接地 150 ms 后开始限速伸缩，最大速度 0.10 m/s。
    ground_samples = min(ground_samples + 1, 150);
    if ground_samples >= 150
        max_step = 0.10 * 0.001;
        if isfinite(L_length_request) && L_length_request > 0
            L_ref = L_ref + max(-max_step, min(max_step, L_length_request - L_ref));
        end
        if isfinite(R_length_request) && R_length_request > 0
            R_ref = R_ref + max(-max_step, min(max_step, R_length_request - R_ref));
        end
    end
else
    ground_samples = 0;
end

L_length_ref = L_ref;
R_length_ref = R_ref;
end

== matlab function blance_leg2_RPY/Subsystem/MATLAB Function5 ==
  data: phi1 input; Z_rel_Dot output; phi4 input; d_phi1 input; d_phi4 input; theta input; d_theta input; valid_speed output
function [Z_rel_Dot, valid_speed] = fcn( ...
    phi1, phi4, d_phi1, d_phi4, theta, d_theta)

[Z_rel_Dot, valid_speed] = wheel_relative_vertical_rate( ...
    phi1, phi4, d_phi1, d_phi4, theta, d_theta);
end

== matlab function blance_leg2_RPY/Subsystem5/MATLAB Function5 ==
  data: phi1 input; Z_rel_Dot output; phi4 input; d_phi1 input; d_phi4 input; theta input; d_theta input; valid_speed output
function [Z_rel_Dot, valid_speed] = fcn( ...
    phi1, phi4, d_phi1, d_phi4, theta, d_theta)

[Z_rel_Dot, valid_speed] = wheel_relative_vertical_rate( ...
    phi1, phi4, d_phi1, d_phi4, theta, d_theta);
end

== matlab function blance_leg2_RPY/Right Wheel Carrier Rate ==
  data: phi1 input; omega output; phi4 input; w1 input; w4 input; bodyPitchRate input
function omega = carrier_world_rate(phi1,phi4,w1,w4,bodyPitchRate)
%#codegen
% 实际轮电机基座（连杆 BC）绕世界 X 轴的角速度，单位 rad/s。
% 输入采用与 control/Subsystem4 和 calc/Subsystem1 相同的坐标约定。
% 几何参数与 VMC_calc 一致，髋轴间距为 100 mm。
l1=0.12; l2=0.18; l3=0.18; l4=0.12; l5=0.10;
xb=l1*cos(phi1); yb=l1*sin(phi1);
xd=l5+l4*cos(phi4); yd=l4*sin(phi4);
a=2*l2*(xd-xb); b=2*l2*(yd-yb);
c=l2*l2+(xd-xb)^2+(yd-yb)^2-l3*l3;
disc=a*a+b*b-c*c;
assert(disc >= -1e-12, 'Unreachable five-bar geometry');
phi2=2*atan2(b+sqrt(max(disc,0)),a+c);
phi3=atan2(yb-yd+l2*sin(phi2),xb-xd+l2*cos(phi2));
den=l2*sin(phi3-phi2);
assert(abs(den)>1e-10, 'Five-bar velocity singularity');
w2=(l1*sin(phi1-phi3)*w1+l4*sin(phi3-phi4)*w4)/den;
% 本模型中，实际连杆转动与机身俯仰角速度在世界 X 轴方向相加。
omega=w2+bodyPitchRate;
end

== matlab function blance_leg2_RPY/Left Wheel Carrier Rate ==
  data: phi1 input; omega output; phi4 input; w1 input; w4 input; bodyPitchRate input
function omega = carrier_world_rate(phi1,phi4,w1,w4,bodyPitchRate)
%#codegen
% 实际轮电机基座（连杆 BC）绕世界 X 轴的角速度，单位 rad/s。
% 输入采用与 control/Subsystem4 和 calc/Subsystem1 相同的坐标约定。
% 几何参数与 VMC_calc 一致，髋轴间距为 100 mm。
l1=0.12; l2=0.18; l3=0.18; l4=0.12; l5=0.10;
xb=l1*cos(phi1); yb=l1*sin(phi1);
xd=l5+l4*cos(phi4); yd=l4*sin(phi4);
a=2*l2*(xd-xb); b=2*l2*(yd-yb);
c=l2*l2+(xd-xb)^2+(yd-yb)^2-l3*l3;
disc=a*a+b*b-c*c;
assert(disc >= -1e-12, 'Unreachable five-bar geometry');
phi2=2*atan2(b+sqrt(max(disc,0)),a+c);
phi3=atan2(yb-yd+l2*sin(phi2),xb-xd+l2*cos(phi2));
den=l2*sin(phi3-phi2);
assert(abs(den)>1e-10, 'Five-bar velocity singularity');
w2=(l1*sin(phi1-phi3)*w1+l4*sin(phi3-phi4)*w4)/den;
% 本模型中，实际连杆转动与机身俯仰角速度在世界 X 轴方向相加。
omega=w2+bodyPitchRate;
end

== matlab function blance_leg2_RPY/Subsystem2/MATLAB Function ==
  settings: updateMethod=DISCRETE  sampleTime=0.001
  data: phi1 input; F_N output; phi4 input; T1 input; T2 input; theta input; Z_M_Ddot input; valid output; Z_rel_Dot input; valid_speed input
function [F_N, valid] = fcn( ...
    phi1, phi4, T1, T2, theta, Z_M_Ddot, Z_rel_Dot, valid_speed)
% 每 1 ms 采样。传力和竖直加速度均对应最近 2 ms。
% 传力先用每一拍的关节状态和力矩单独解算，再做梯形平均。
persistent acc_history speed_history force_history valid_history
if isempty(valid_history)
    acc_history = zeros(2,1);
    speed_history = zeros(2,1);
    force_history = zeros(2,1);
    valid_history = false(2,1);
end

motion_valid = valid_speed && isfinite(Z_M_Ddot) && isfinite(Z_rel_Dot);
window_valid = motion_valid && all(valid_history);
Z_M_Ddot_avg = 0;
Z_rel_Ddot = 0;
if window_valid
    Z_M_Ddot_avg = (acc_history(1) + 2*acc_history(2) + Z_M_Ddot) / 4;
    Z_rel_Ddot = (Z_rel_Dot - speed_history(1)) / 0.002;
end

[F_instant_P, force_valid, P_now] = estimate_support_force_rm( ...
    phi1, phi4, T1, T2, theta, Z_M_Ddot_avg, Z_rel_Ddot);
sample_valid = motion_valid && force_valid && isfinite(F_instant_P) && isfinite(P_now);
valid = window_valid && sample_valid;
F_N = NaN;
if valid
    P_avg = (force_history(1) + 2*force_history(2) + P_now) / 4;
    % 轮子的惯性项已经对应同一窗口，只替换腿部传力项。
    F_N = (F_instant_P - P_now) + P_avg;
end

acc_history = [acc_history(2); Z_M_Ddot];
speed_history = [speed_history(2); Z_rel_Dot];
force_history = [force_history(2); P_now];
valid_history = [valid_history(2); sample_valid];
end

== matlab function blance_leg2_RPY/Subsystem3/MATLAB Function ==
  settings: updateMethod=DISCRETE  sampleTime=0.001
  data: phi1 input; F_N output; phi4 input; T1 input; T2 input; theta input; Z_M_Ddot input; valid output; Z_rel_Dot input; valid_speed input
function [F_N, valid] = fcn( ...
    phi1, phi4, T1, T2, theta, Z_M_Ddot, Z_rel_Dot, valid_speed)
% 每 1 ms 采样。传力和竖直加速度均对应最近 2 ms。
% 传力先用每一拍的关节状态和力矩单独解算，再做梯形平均。
persistent acc_history speed_history force_history valid_history
if isempty(valid_history)
    acc_history = zeros(2,1);
    speed_history = zeros(2,1);
    force_history = zeros(2,1);
    valid_history = false(2,1);
end

motion_valid = valid_speed && isfinite(Z_M_Ddot) && isfinite(Z_rel_Dot);
window_valid = motion_valid && all(valid_history);
Z_M_Ddot_avg = 0;
Z_rel_Ddot = 0;
if window_valid
    Z_M_Ddot_avg = (acc_history(1) + 2*acc_history(2) + Z_M_Ddot) / 4;
    Z_rel_Ddot = (Z_rel_Dot - speed_history(1)) / 0.002;
end

[F_instant_P, force_valid, P_now] = estimate_support_force_rm( ...
    phi1, phi4, T1, T2, theta, Z_M_Ddot_avg, Z_rel_Ddot);
sample_valid = motion_valid && force_valid && isfinite(F_instant_P) && isfinite(P_now);
valid = window_valid && sample_valid;
F_N = NaN;
if valid
    P_avg = (force_history(1) + 2*force_history(2) + P_now) / 4;
    % 轮子的惯性项已经对应同一窗口，只替换腿部传力项。
    F_N = (F_instant_P - P_now) + P_avg;
end

acc_history = [acc_history(2); Z_M_Ddot];
speed_history = [speed_history(2); Z_rel_Dot];
force_history = [force_history(2); P_now];
valid_history = [valid_history(2); sample_valid];
end

== matlab function blance_leg2_RPY/MATLAB Function2 ==
  settings: updateMethod=DISCRETE  sampleTime=0.001
  data: F_N_L input; T_air output; F_N_R input; valid_L input; valid_R input; PITCH input; d_PITCH input; on_ground output
function [T_air, on_ground] = fcn( ...
    F_N_L, F_N_R, valid_L, valid_R, PITCH, d_PITCH)

[T_air, on_ground] = airborne_pitch_mode( ...
    F_N_L, F_N_R, valid_L, valid_R, PITCH, d_PITCH);
end

== matlab function blance_leg2_RPY/MATLAB Function3 ==
  data: on_ground input; L_T_cmd output; T_air input; L_T_ground input; R_T_ground input; R_T_cmd output
function [L_T_cmd, R_T_cmd] = fcn(on_ground, T_air, L_T_ground, R_T_ground)
    if on_ground
        L_T_cmd = L_T_ground;
        R_T_cmd = R_T_ground;
    else
        L_T_cmd = T_air;
        R_T_cmd = T_air;
    end
end

== matlab function blance_leg2_RPY/Subsystem4/MATLAB Function10 ==
  data: L0 output; phi1 input; phi4 input; phi0 output
function [L0,phi0] = fcn(phi1,phi4)
   
    l5=0.10;%AE长度
    l1=0.12;
    l2=0.18;
    l3=0.18;
    l4=0.12;
    
    YD = l4*sin(phi4);
    YB = l1*sin(phi1);
    XD = l5 + l4*cos(phi4);
    XB = l1*cos(phi1); 
    lBD = sqrt((XD - XB)*(XD - XB) + (YD - YB)*(YD - YB));
    A0 = 2*l2*(XD - XB);
    B0 = 2*l2*(YD - YB);
    C0 = l2*l2 + lBD*lBD - l3*l3;
    phi2 = 2*atan2((B0 + sqrt(A0*A0 + B0*B0 - C0*C0)),(A0 + C0));
    XC = l1*cos(phi1) + l2*cos(phi2);
    YC = l1*sin(phi1) + l2*sin(phi2);
    L0 = sqrt((XC - l5/2)*(XC - l5/2) + YC*YC);
    phi0=atan2(YC,(XC-l5/2));
    
end
